simulink library "fuselage_lib"  (R2018b)
settings: Solver=VariableStepAuto  StartTime=0.0  StopTime=10.0  RelTol=1e-3
undefined symbols (not defined in the file or in its folder): fuselage_state_bus, fuselage_struct
libraries: $bdroot x4
settings Model: Creator=Ybeyer  LastModifiedBy=yannic
settings SFSimCC: SimUseLocalCustomCode=off
settings RTWCC: RTWUseLocalCustomCode=off
settings CodeAppCC: StateflowObjectComments=on

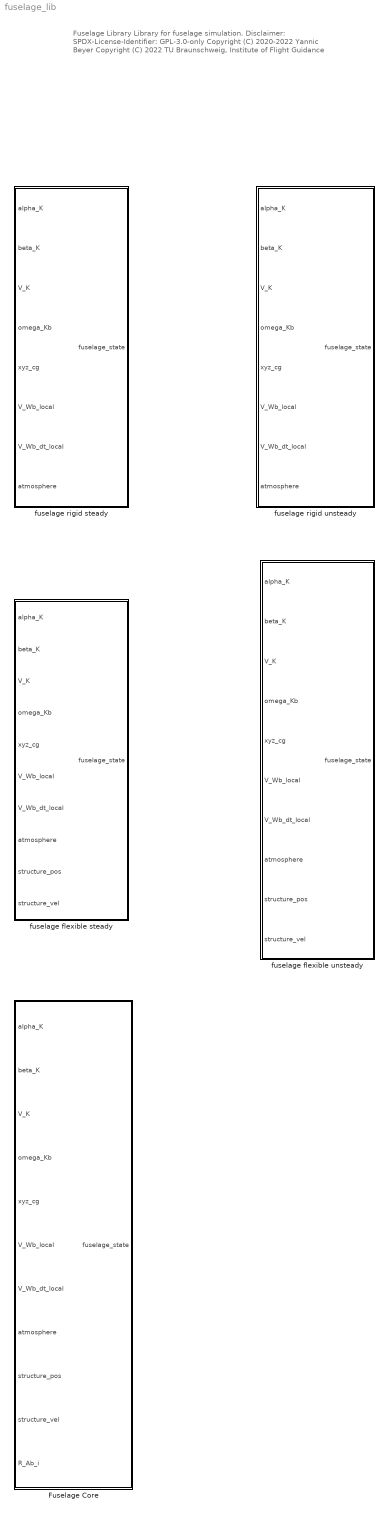
== system fuselage_lib ==
  note: Fuselage Library
      |
      | Library for fuselage simulation.
      |
      | Disclaimer:
      | SPDX-License-Identifier: GPL-3.0-only
      |
      | Copyright (C) 2020-2022 Yannic Beyer
      | Copyright (C) 2022 TU Braunschweig, Institute of Flight Guidance
  Fuselage Core : Subsystem  mask{fuselage_struct=fuselage_struct, fuselage_state_bus=fuselage_state_bus}
      mask prompts: fuselage_struct "Fuselage struct"; fuselage_state_bus "Fuselage state bus"
      mask DialogControl DescGroupVar Prompt: Fuselage Core
  fuselage flexible steady : Subsystem  mask{fuselage_struct=fuselage_struct, fuselage_state_bus=fuselage_state_bus}
      mask prompts: fuselage_struct "Fuselage struct"; fuselage_state_bus "Fuselage state bus"
      mask DialogControl DescGroupVar Prompt: Discretized fuselage aerodynamics (rigid)
      mask DialogControl DescTextVar Prompt: This block computes the aerodynamics of a fuselage along the centerline. It is based on basic methods.
      mask DialogControl Control2 Prompt: The inputs and outputs are described in the README:
      mask DialogControl Control3 Prompt: README
      mask DialogControl Control3 Callback: web('https://github.com/iff-gsc/ladac/-/blob/master/aerodynamics/fuselage/README.md','-browser')
      mask DialogControl Control4 Prompt: To initialize a fuselage struct, please use the function fuselageCreate.
      mask DialogControl Control5 Prompt: The fuselage state bus can then be created by running fuselage_state_bus = struct2bus_(fuselage.state)
  fuselage flexible unsteady : Subsystem  mask{fuselage_struct=fuselage_struct, fuselage_state_bus=fuselage_state_bus}
      mask prompts: fuselage_struct "Fuselage struct"; fuselage_state_bus "Fuselage state bus"
      mask DialogControl DescGroupVar Prompt: Discretized fuselage aerodynamics (aeroelastic)
      mask DialogControl DescTextVar Prompt: This block computes the aerodynamics of a fuselage along the centerline. It is based on basic methods.
      mask DialogControl Control2 Prompt: The inputs and outputs are described in the README:
      mask DialogControl Control3 Prompt: README
      mask DialogControl Control3 Callback: web('https://github.com/iff-gsc/ladac/-/blob/master/aerodynamics/fuselage/README.md','-browser')
      mask DialogControl Control4 Prompt: To initialize a fuselage struct, please use the function fuselageCreate.
      mask DialogControl Control5 Prompt: The fuselage state bus can then be created by running fuselage_state_bus = struct2bus_(fuselage.state)
  fuselage rigid steady : Subsystem  mask{fuselage_struct=fuselage_struct, fuselage_state_bus=fuselage_state_bus}
      mask prompts: fuselage_struct "Fuselage struct"; fuselage_state_bus "Fuselage state bus"
      mask DialogControl DescGroupVar Prompt: Discretized fuselage aerodynamics (rigid)
      mask DialogControl DescTextVar Prompt: This block computes the aerodynamics of a fuselage along the centerline. It is based on basic methods.
      mask DialogControl Control2 Prompt: The inputs and outputs are described in the README:
      mask DialogControl Control3 Prompt: README
      mask DialogControl Control3 Callback: web('https://github.com/iff-gsc/ladac/-/blob/master/aerodynamics/fuselage/README.md','-browser')
      mask DialogControl Control4 Prompt: To initialize a fuselage struct, please use the function fuselageCreate.
      mask DialogControl Control5 Prompt: The fuselage state bus can then be created by running fuselage_state_bus = struct2bus_(fuselage.state)
  fuselage rigid unsteady : Subsystem  mask{fuselage_struct=fuselage_struct, fuselage_state_bus=fuselage_state_bus}
      mask prompts: fuselage_struct "Fuselage struct"; fuselage_state_bus "Fuselage state bus"
      mask DialogControl DescGroupVar Prompt: Discretized fuselage aerodynamics (aeroelastic)
      mask DialogControl DescTextVar Prompt: This block computes the aerodynamics of a fuselage along the centerline. It is based on basic methods.
      mask DialogControl Control2 Prompt: The inputs and outputs are described in the README:
      mask DialogControl Control3 Prompt: README
      mask DialogControl Control3 Callback: web('https://github.com/iff-gsc/ladac/-/blob/master/aerodynamics/fuselage/README.md','-browser')
      mask DialogControl Control4 Prompt: To initialize a fuselage struct, please use the function fuselageCreate.
      mask DialogControl Control5 Prompt: The fuselage state bus can then be created by running fuselage_state_bus = struct2bus_(fuselage.state)

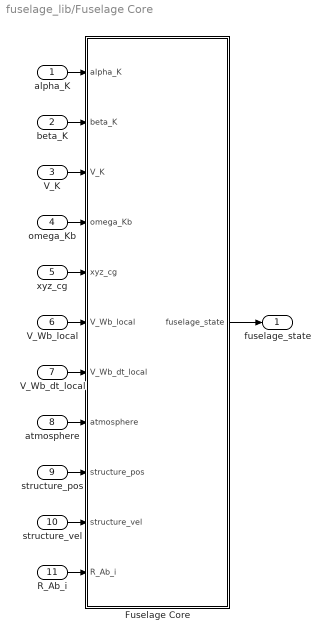
== system fuselage_lib/Fuselage Core ==
  alpha_K : Inport
  beta_K : Inport  Port=2
  V_K : Inport  Port=3
  omega_Kb : Inport  Port=4
  xyz_cg : Inport  Port=5
  V_Wb_local : Inport  Port=6
  V_Wb_dt_local : Inport  Port=7
  atmosphere : Inport  Port=8
  structure_pos : Inport  Port=9
  structure_vel : Inport  Port=10
  R_Ab_i : Inport  Port=11
  Fuselage Core : MATLAB Function  TreatAsAtomicUnit=on
  fuselage_state : Outport
  wires:
  beta_K/1 -> Fuselage Core/2(beta_K)
  Fuselage Core/1(fuselage_state) -> fuselage_state/1
  V_K/1 -> Fuselage Core/3(V_K)
  alpha_K/1 -> Fuselage Core/1(alpha_K)
  omega_Kb/1 -> Fuselage Core/4(omega_Kb)
  xyz_cg/1 -> Fuselage Core/5(xyz_cg)
  atmosphere/1 -> Fuselage Core/8(atmosphere)
  V_Wb_local/1 -> Fuselage Core/6(V_Wb_local)
  V_Wb_dt_local/1 -> Fuselage Core/7(V_Wb_dt_local)
  R_Ab_i/1 -> Fuselage Core/11(R_Ab_i)
  structure_pos/1 -> Fuselage Core/9(structure_pos)
  structure_vel/1 -> Fuselage Core/10(structure_vel)

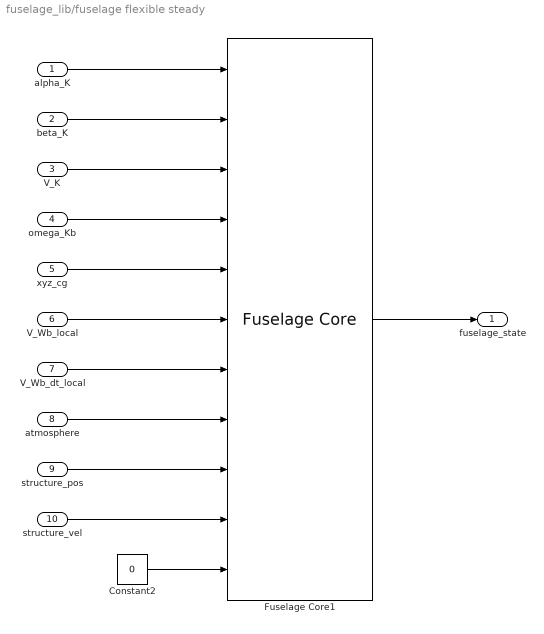
== system fuselage_lib/fuselage flexible steady ==
  alpha_K : Inport
  beta_K : Inport  Port=2
  V_K : Inport  Port=3
  omega_Kb : Inport  Port=4
  xyz_cg : Inport  Port=5
  V_Wb_local : Inport  Port=6
  V_Wb_dt_local : Inport  Port=7
  atmosphere : Inport  Port=8
  structure_pos : Inport  Port=9
  structure_vel : Inport  Port=10
  Constant2 : Constant  Value=0
  Fuselage Core1 : $bdroot/Fuselage Core  fuselage_struct=fuselage_struct  fuselage_state_bus=fuselage_state_bus
  fuselage_state : Outport
  wires:
  Constant2/1 -> Fuselage Core1/11
  V_Wb_local/1 -> Fuselage Core1/6
  atmosphere/1 -> Fuselage Core1/8
  omega_Kb/1 -> Fuselage Core1/4
  V_K/1 -> Fuselage Core1/3
  V_Wb_dt_local/1 -> Fuselage Core1/7
  xyz_cg/1 -> Fuselage Core1/5
  beta_K/1 -> Fuselage Core1/2
  Fuselage Core1/1 -> fuselage_state/1
  alpha_K/1 -> Fuselage Core1/1
  structure_vel/1 -> Fuselage Core1/10
  structure_pos/1 -> Fuselage Core1/9

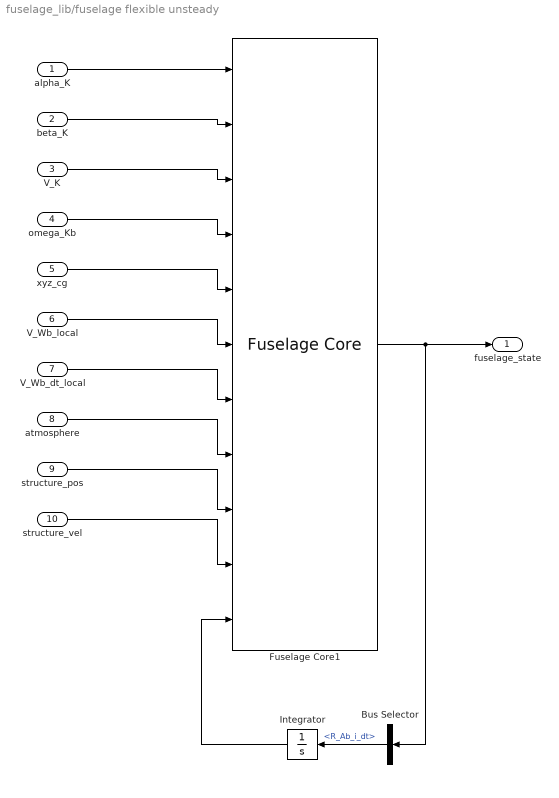
== system fuselage_lib/fuselage flexible unsteady ==
  alpha_K : Inport
  beta_K : Inport  Port=2
  V_K : Inport  Port=3
  omega_Kb : Inport  Port=4
  xyz_cg : Inport  Port=5
  V_Wb_local : Inport  Port=6
  V_Wb_dt_local : Inport  Port=7
  atmosphere : Inport  Port=8
  structure_pos : Inport  Port=9
  structure_vel : Inport  Port=10
  Bus Selector : BusSelector  OutputSignals=aero.R_Ab_i_dt
  Fuselage Core1 : $bdroot/Fuselage Core  fuselage_struct=fuselage_struct  fuselage_state_bus=fuselage_state_bus
  Integrator : Integrator
  fuselage_state : Outport
  wires:
  Fuselage Core1/1 -> fuselage_state/1, Bus Selector/1
  alpha_K/1 -> Fuselage Core1/1
  beta_K/1 -> Fuselage Core1/2
  V_K/1 -> Fuselage Core1/3
  omega_Kb/1 -> Fuselage Core1/4
  xyz_cg/1 -> Fuselage Core1/5
  V_Wb_local/1 -> Fuselage Core1/6
  V_Wb_dt_local/1 -> Fuselage Core1/7
  atmosphere/1 -> Fuselage Core1/8
  structure_pos/1 -> Fuselage Core1/9
  structure_vel/1 -> Fuselage Core1/10
  Bus Selector/1 -> Integrator/1  "<R_Ab_i_dt>"
  Integrator/1 -> Fuselage Core1/11

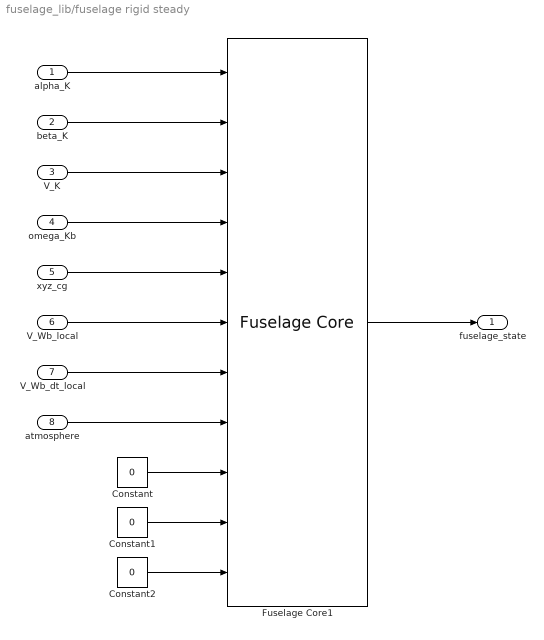
== system fuselage_lib/fuselage rigid steady ==
  alpha_K : Inport
  beta_K : Inport  Port=2
  V_K : Inport  Port=3
  omega_Kb : Inport  Port=4
  xyz_cg : Inport  Port=5
  V_Wb_local : Inport  Port=6
  V_Wb_dt_local : Inport  Port=7
  atmosphere : Inport  Port=8
  Constant : Constant  Value=0
  Constant1 : Constant  Value=0
  Constant2 : Constant  Value=0
  Fuselage Core1 : $bdroot/Fuselage Core  fuselage_struct=fuselage_struct  fuselage_state_bus=fuselage_state_bus
  fuselage_state : Outport
  wires:
  alpha_K/1 -> Fuselage Core1/1
  Fuselage Core1/1 -> fuselage_state/1
  beta_K/1 -> Fuselage Core1/2
  xyz_cg/1 -> Fuselage Core1/5
  V_Wb_dt_local/1 -> Fuselage Core1/7
  V_K/1 -> Fuselage Core1/3
  omega_Kb/1 -> Fuselage Core1/4
  atmosphere/1 -> Fuselage Core1/8
  V_Wb_local/1 -> Fuselage Core1/6
  Constant/1 -> Fuselage Core1/9
  Constant1/1 -> Fuselage Core1/10
  Constant2/1 -> Fuselage Core1/11

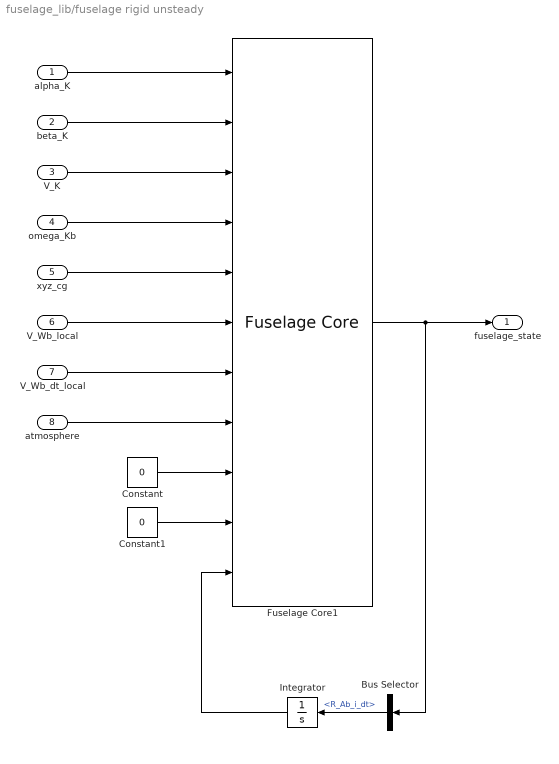
== system fuselage_lib/fuselage rigid unsteady ==
  alpha_K : Inport
  beta_K : Inport  Port=2
  V_K : Inport  Port=3
  omega_Kb : Inport  Port=4
  xyz_cg : Inport  Port=5
  V_Wb_local : Inport  Port=6
  V_Wb_dt_local : Inport  Port=7
  atmosphere : Inport  Port=8
  Bus Selector : BusSelector  OutputSignals=aero.R_Ab_i_dt
  Constant : Constant  Value=0
  Constant1 : Constant  Value=0
  Fuselage Core1 : $bdroot/Fuselage Core  fuselage_struct=fuselage_struct  fuselage_state_bus=fuselage_state_bus
  Integrator : Integrator
  fuselage_state : Outport
  wires:
  Integrator/1 -> Fuselage Core1/11
  Bus Selector/1 -> Integrator/1  "<R_Ab_i_dt>"
  atmosphere/1 -> Fuselage Core1/8
  V_Wb_dt_local/1 -> Fuselage Core1/7
  V_Wb_local/1 -> Fuselage Core1/6
  xyz_cg/1 -> Fuselage Core1/5
  omega_Kb/1 -> Fuselage Core1/4
  V_K/1 -> Fuselage Core1/3
  beta_K/1 -> Fuselage Core1/2
  alpha_K/1 -> Fuselage Core1/1
  Fuselage Core1/1 -> Bus Selector/1, fuselage_state/1
  Constant1/1 -> Fuselage Core1/10
  Constant/1 -> Fuselage Core1/9

== matlab function fuselage_lib/Fuselage Core/Fuselage Core ==
  data: fuselage_state output fuselage_state_bus; alpha_K input; beta_K input; V_K input; omega_Kb input; xyz_cg input; V_Wb_local input; V_Wb_dt_local input; atmosphere input; structure_pos input; structure_vel input; R_Ab_i input; fuselage_struct parameter
function fuselage_state = fuselageCore(alpha_K,beta_K,V_K,...
    omega_Kb,xyz_cg,V_Wb_local,V_Wb_dt_local,atmosphere,...
    structure_pos,structure_vel,R_Ab_i, fuselage_struct)

% compute and set fuselage state
fuselage_struct = fuselageSetState( fuselage_struct, alpha_K, beta_K, V_K, omega_Kb, ...
    xyz_cg, 'atmosphere', atmosphere, 'V_Wb', V_Wb_local, 'V_Wb_dt', V_Wb_dt_local, ...
    'structure_pos', structure_pos, 'structure_vel', structure_vel, ...
    'unsteady', R_Ab_i );

% function output is only the state (the rest is constant - except of
% fuselage.external)
fuselage_state = fuselage_struct.state;

end
